simulink model "uartDemo"  (R2023a)
settings: Solver=ode4  StartTime=0.0  StopTime=0.011  FixedStep=0.01  RelTol=1e-3
libraries: simulink x10, instrumentseriallib x4, slrealtimeutilitieslib x2, svdutilitieslib x1
settings Model: Creator=zhuxh  LastModifiedBy=zqinghua
settings SolverCC: AlgebraicLoopSolver=TrustRegion
settings DebuggingCC: ArithmeticOperatorsInVariantConditions=warning
settings SFSimCC: CustomCodeUndefinedFunction=UseInterfaceOnly
settings CodeAppCC: StateflowObjectComments=on

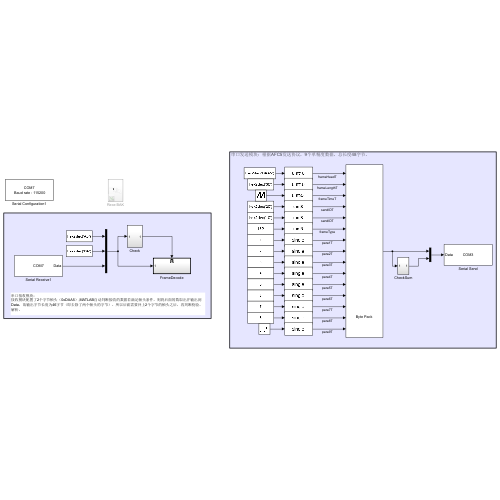
[thumbnail: Simulink's stored preview of the top-level diagram]
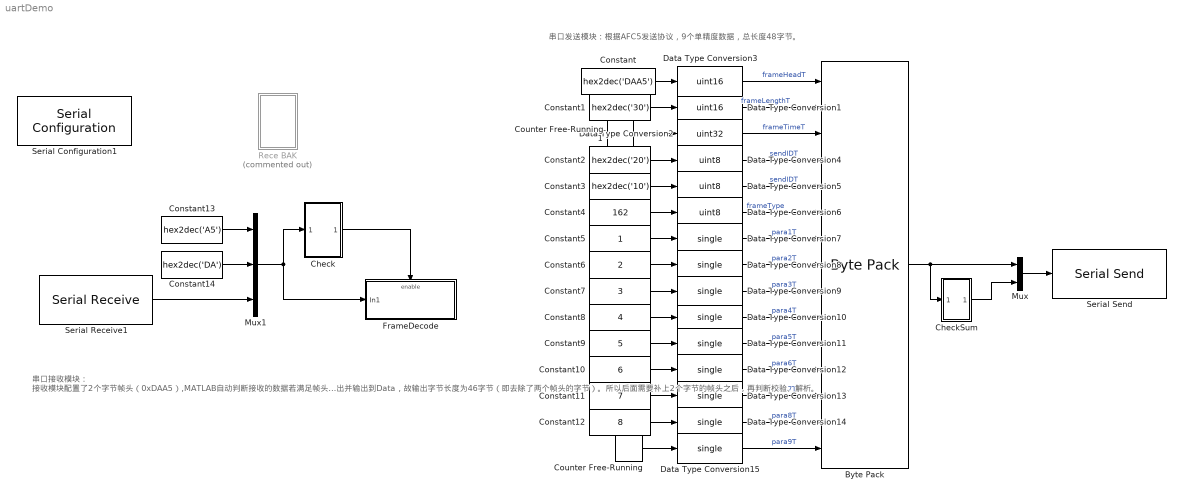
== system uartDemo ==
  note: 串口发送模块：根据AFC5发送协议，9个单精度数据，总长度48字节。
  note: 串口接收模块：
      | 接收模块配置了2个字节帧头（0xDAA5）,MATLAB自动判断接收的数据若满足帧头条件，则将后面的数取出并输出到Data，故输出字节长度为46字节（即去除了两个帧头的字节）。所以后面需要补上2个字节的帧头之后，再判断校验、解析。
  Byte Pack : svdutilitieslib/Byte Pack  maskPackedDataType=uint8  datatypes={'uint16','uint16','uint32','uint8','uint8','uint8','single','single','single','single','single','single','single','single','single'}  byteAlign=1  blockPlatform=tic2000
      settings: LibrarySourceBlock=c2000lib/Target Communication/Byte Pack
  Check : Subsystem
  CheckSum : Subsystem
  Constant : Constant  Value=hex2dec('DAA5')  SampleTime=-1
  Constant1 : Constant  Value=hex2dec('30')  SampleTime=-1
  Constant10 : Constant  Value=6  SampleTime=-1
  Constant11 : Constant  Value=7  SampleTime=-1
  Constant12 : Constant  Value=8  SampleTime=-1
  Constant13 : Constant  Value=hex2dec('A5')  OutDataTypeStr=uint8  SampleTime=-1
  Constant14 : Constant  Value=hex2dec('DA')  OutDataTypeStr=uint8  SampleTime=-1
  Constant2 : Constant  Value=hex2dec('20')  SampleTime=-1
  Constant3 : Constant  Value=hex2dec('10')  SampleTime=-1
  Constant4 : Constant  Value=162  SampleTime=-1
  Constant5 : Constant  SampleTime=-1
  Constant6 : Constant  Value=2  SampleTime=-1
  Constant7 : Constant  Value=3  SampleTime=-1
  Constant8 : Constant  Value=4  SampleTime=-1
  Constant9 : Constant  Value=5  SampleTime=-1
  Counter Free-Running : simulink/Sources/Counter Free-Running  NumBits=32  tsamp=-1
  Counter Free-Running1 : simulink/Sources/Counter Free-Running  NumBits=32  tsamp=-1
  Data Type Conversion1 : DataTypeConversion  OutDataTypeStr=uint16  SaturateOnIntegerOverflow=off  RndMeth=Floor
  Data Type Conversion{7..15} (9 alike) : DataTypeConversion  OutDataTypeStr=single  SaturateOnIntegerOverflow=off  RndMeth=Floor
  Data Type Conversion2 : DataTypeConversion  OutDataTypeStr=uint32  SaturateOnIntegerOverflow=off  RndMeth=Floor
  Data Type Conversion3 : DataTypeConversion  OutDataTypeStr=uint16  SaturateOnIntegerOverflow=off  RndMeth=Floor
  Data Type Conversion4 : DataTypeConversion  OutDataTypeStr=uint8  SaturateOnIntegerOverflow=off  RndMeth=Floor
  Data Type Conversion5 : DataTypeConversion  OutDataTypeStr=uint8  SaturateOnIntegerOverflow=off  RndMeth=Floor
  Data Type Conversion6 : DataTypeConversion  OutDataTypeStr=uint8  SaturateOnIntegerOverflow=off  RndMeth=Floor
  FrameDecode : Subsystem  TreatAsAtomicUnit=on
  Mux : Mux  Inputs=2
  Mux1 : Mux  Inputs=3
  Rece BAK : Subsystem  Commented=on
  Serial Configuration1 : instrumentseriallib/Serial Configuration  Priority=-200000  PortSel=COM7  Port=COM7  ComPort=COM7  BaudRate=115200  DataBits=8  Parity=none  StopBits=1  ByteOrder=little-endian  FlowControl=none  Timeout=10  SimulateUsing=Interpreted execution  BlockInModel=on  aMode=1
  Serial Receive1 : instrumentseriallib/Serial Receive  Priority=1  PortSel=COM7  Port=COM7  ComPort=COM7  DataType=uint8  SaveDataType=uint8  ToggleHeader=on  Header=[hex2dec('DA') hex2dec('A5')]  ToggleTerminator=off  Terminator=<none>  CustomTerminator=[]  InputFormat=Column major  ToggleDataSize=on  DataSize=46  EnableBlockingMode=on  ActionDataUnavailable=Output last received value  ActionWhenDataUnavailable=Output last received value  CustomValue=0  SampleTime=-1  SimulateUsing=Interpreted execution  BlockInModel=on  aMode=1
  Serial Send : instrumentseriallib/Serial Send  Priority=1  PortSel=COM3  Port=COM3  ComPort=COM3  Header=[]  Terminator=<none>  CustomTerminator=[]  EnableBlockingMode=on  SimulateUsing=Interpreted execution  BlockInModel=on  aMode=1
  wires:
  Data Type Conversion4/1 -> Byte Pack/4  "sendIDT"
  Data Type Conversion5/1 -> Byte Pack/5  "sendIDT"
  Data Type Conversion8/1 -> Byte Pack/8  "para2T"
  Data Type Conversion3/1 -> Byte Pack/1  "frameHeadT"
  Constant5/1 -> Data Type Conversion7/1
  Constant8/1 -> Data Type Conversion10/1
  Constant6/1 -> Data Type Conversion8/1
  Data Type Conversion11/1 -> Byte Pack/11  "para5T"
  Constant11/1 -> Data Type Conversion13/1
  Data Type Conversion10/1 -> Byte Pack/10  "para4T"
  Constant10/1 -> Data Type Conversion12/1
  Constant7/1 -> Data Type Conversion9/1
  Data Type Conversion7/1 -> Byte Pack/7  "para1T"
  Constant2/1 -> Data Type Conversion4/1
  Counter Free-Running1/1 -> Data Type Conversion2/1
  Mux/1 -> Serial Send/1
  Data Type Conversion2/1 -> Byte Pack/3  "frameTimeT"
  Counter Free-Running/1 -> Data Type Conversion15/1
  Data Type Conversion13/1 -> Byte Pack/13  "para7T"
  Data Type Conversion6/1 -> Byte Pack/6  "frameType"
  Data Type Conversion9/1 -> Byte Pack/9  "para3T"
  Constant/1 -> Data Type Conversion3/1
  Constant12/1 -> Data Type Conversion14/1
  Constant9/1 -> Data Type Conversion11/1
  CheckSum/1(Out1) -> Mux/2
  Data Type Conversion12/1 -> Byte Pack/12  "para6T"
  Constant4/1 -> Data Type Conversion6/1
  Data Type Conversion15/1 -> Byte Pack/15  "para9T"
  Constant1/1 -> Data Type Conversion1/1
  Constant3/1 -> Data Type Conversion5/1
  Data Type Conversion14/1 -> Byte Pack/14  "para8T"
  Byte Pack/1 -> CheckSum/1(In1), Mux/1
  Data Type Conversion1/1 -> Byte Pack/2  "frameLengthT"
  Serial Receive1/1 -> Mux1/3
  Constant13/1 -> Mux1/1
  Constant14/1 -> Mux1/2
  Mux1/1 -> Check/1(In1), FrameDecode/1(In1)
  Check/1(Out1) -> FrameDecode/Enable

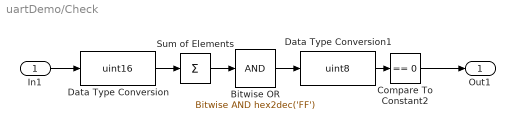
== system uartDemo/Check ==
  In1 : Inport
  Bitwise OR : simulink/Logic and Bit Operations/Bitwise Operator  logicop=AND  UseBitMask=on  BitMask=hex2dec('FF')  BitMaskRealWorld=Stored Integer
  Compare To Constant2 : simulink/Logic and Bit Operations/Compare To Constant  relop===  const=0  OutDataTypeStr=boolean
  Data Type Conversion : DataTypeConversion  OutDataTypeStr=uint16  SaturateOnIntegerOverflow=off  RndMeth=Floor
  Data Type Conversion1 : DataTypeConversion  OutDataTypeStr=uint8  SaturateOnIntegerOverflow=off  RndMeth=Floor
  Sum of Elements : Sum  Inputs=+
  Out1 : Outport
  wires:
  Compare To Constant2/1 -> Out1/1
  Sum of Elements/1 -> Bitwise OR/1
  Bitwise OR/1 -> Data Type Conversion1/1
  Data Type Conversion/1 -> Sum of Elements/1
  Data Type Conversion1/1 -> Compare To Constant2/1
  In1/1 -> Data Type Conversion/1

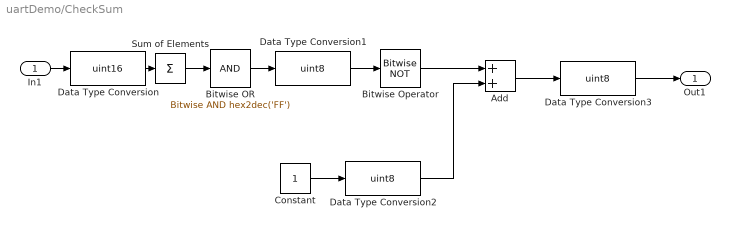
== system uartDemo/CheckSum ==
  In1 : Inport
  Add : Sum
  Bitwise Operator : simulink/Logic and Bit Operations/Bitwise Operator  logicop=NOT  UseBitMask=off  BitMask=bin2dec('11011001')  BitMaskRealWorld=Stored Integer
  Bitwise OR : simulink/Logic and Bit Operations/Bitwise Operator  logicop=AND  UseBitMask=on  BitMask=hex2dec('FF')  BitMaskRealWorld=Stored Integer
  Constant : Constant
  Data Type Conversion : DataTypeConversion  OutDataTypeStr=uint16  SaturateOnIntegerOverflow=off  RndMeth=Floor
  Data Type Conversion1 : DataTypeConversion  OutDataTypeStr=uint8  SaturateOnIntegerOverflow=off  RndMeth=Floor
  Data Type Conversion2 : DataTypeConversion  OutDataTypeStr=uint8  SaturateOnIntegerOverflow=off  RndMeth=Floor
  Data Type Conversion3 : DataTypeConversion  OutDataTypeStr=uint8  SaturateOnIntegerOverflow=off  RndMeth=Floor
  Sum of Elements : Sum  Inputs=+
  Out1 : Outport
  wires:
  Data Type Conversion3/1 -> Out1/1
  Sum of Elements/1 -> Bitwise OR/1
  Bitwise OR/1 -> Data Type Conversion1/1
  Data Type Conversion/1 -> Sum of Elements/1
  Data Type Conversion1/1 -> Bitwise Operator/1
  In1/1 -> Data Type Conversion/1
  Bitwise Operator/1 -> Add/1
  Constant/1 -> Data Type Conversion2/1
  Data Type Conversion2/1 -> Add/2
  Add/1 -> Data Type Conversion3/1

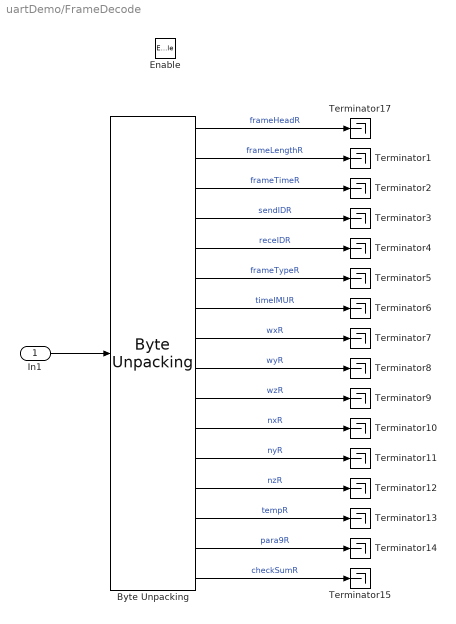
== system uartDemo/FrameDecode ==
  In1 : Inport
  Enable : EnablePort
  "Byte Unpacking " : slrealtimeutilitieslib/Byte Unpacking  MaskUnpackedDataTypes={'uint16','uint16','uint32','uint8','uint8','uint8','single','single','single','single','single','single','single','single','single','uint8'}  MaskUnpackedDataSizes={1,1,1,1,1,1,1,1,1,1,1,1,1,1,1,1}  MaskAlignment=1
  Terminator{1..15,17} (16 alike) : Terminator
  wires:
  "Byte Unpacking "/11 -> Terminator10/1  "nxR"
  "Byte Unpacking "/1 -> Terminator17/1  "frameHeadR"
  "Byte Unpacking "/8 -> Terminator7/1  "wxR"
  "Byte Unpacking "/13 -> Terminator12/1  "nzR"
  "Byte Unpacking "/5 -> Terminator4/1  "receIDR"
  "Byte Unpacking "/14 -> Terminator13/1  "tempR"
  "Byte Unpacking "/6 -> Terminator5/1  "frameTypeR"
  "Byte Unpacking "/3 -> Terminator2/1  "frameTimeR"
  "Byte Unpacking "/2 -> Terminator1/1  "frameLengthR"
  "Byte Unpacking "/16 -> Terminator15/1  "checkSumR"
  "Byte Unpacking "/15 -> Terminator14/1  "para9R"
  "Byte Unpacking "/12 -> Terminator11/1  "nyR"
  "Byte Unpacking "/10 -> Terminator9/1  "wzR"
  "Byte Unpacking "/9 -> Terminator8/1  "wyR"
  "Byte Unpacking "/7 -> Terminator6/1  "timeIMUR"
  "Byte Unpacking "/4 -> Terminator3/1  "sendIDR"
  In1/1 -> "Byte Unpacking "/1

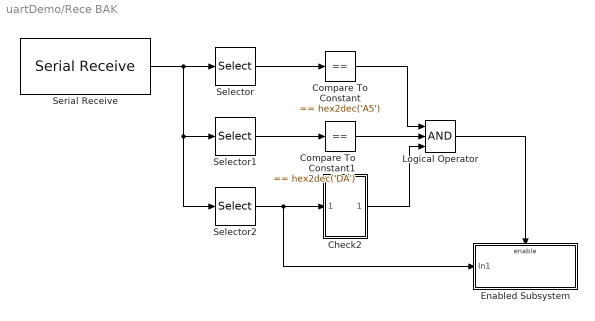
== system uartDemo/Rece BAK ==
  Check2 : Subsystem
  Compare To Constant : simulink/Logic and Bit Operations/Compare To Constant  relop===  const=hex2dec('A5')  OutDataTypeStr=boolean
  Compare To Constant1 : simulink/Logic and Bit Operations/Compare To Constant  relop===  const=hex2dec('DA')  OutDataTypeStr=boolean
  Enabled Subsystem : Subsystem  TreatAsAtomicUnit=on
  Logical Operator : Logic  Inputs=3  AllPortsSameDT=off  OutDataTypeStr=boolean
  Selector : Selector  InputPortWidth=48  IndexOptions=Index vector (dialog)  Indices=[1]  OutputSizes=1
  Selector1 : Selector  InputPortWidth=48  IndexOptions=Index vector (dialog)  Indices=[2]  OutputSizes=1
  Selector2 : Selector  InputPortWidth=48  IndexOptions=Index vector (dialog)  Indices=[1:48]  OutputSizes=1
  Serial Receive : instrumentseriallib/Serial Receive  Priority=1  PortSel=COM3  Port=COM3  ComPort=COM3  DataType=uint8  SaveDataType=uint8  ToggleHeader=off  Header=[]  ToggleTerminator=off  Terminator=<none>  CustomTerminator=[]  InputFormat=Column major  ToggleDataSize=on  DataSize=48  EnableBlockingMode=on  ActionDataUnavailable=Output last received value  ActionWhenDataUnavailable=Output last received value  CustomValue=0  SampleTime=-1  SimulateUsing=Interpreted execution  BlockInModel=on  aMode=1
  wires:
  Logical Operator/1 -> Enabled Subsystem/Enable
  Serial Receive/1 -> Selector/1, Selector2/1, Selector1/1
  Check2/1(Out1) -> Logical Operator/3
  Selector1/1 -> Compare To Constant1/1
  Selector/1 -> Compare To Constant/1
  Compare To Constant/1 -> Logical Operator/1
  Compare To Constant1/1 -> Logical Operator/2
  Selector2/1 -> Enabled Subsystem/1(In1), Check2/1(In1)

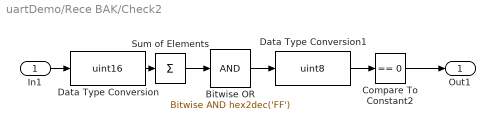
== system uartDemo/Rece BAK/Check2 ==
  In1 : Inport
  Bitwise OR : simulink/Logic and Bit Operations/Bitwise Operator  logicop=AND  UseBitMask=on  BitMask=hex2dec('FF')  BitMaskRealWorld=Stored Integer
  Compare To Constant2 : simulink/Logic and Bit Operations/Compare To Constant  relop===  const=0  OutDataTypeStr=boolean
  Data Type Conversion : DataTypeConversion  OutDataTypeStr=uint16  SaturateOnIntegerOverflow=off  RndMeth=Floor
  Data Type Conversion1 : DataTypeConversion  OutDataTypeStr=uint8  SaturateOnIntegerOverflow=off  RndMeth=Floor
  Sum of Elements : Sum  Inputs=+
  Out1 : Outport
  wires:
  Compare To Constant2/1 -> Out1/1
  Sum of Elements/1 -> Bitwise OR/1
  Bitwise OR/1 -> Data Type Conversion1/1
  Data Type Conversion/1 -> Sum of Elements/1
  Data Type Conversion1/1 -> Compare To Constant2/1
  In1/1 -> Data Type Conversion/1

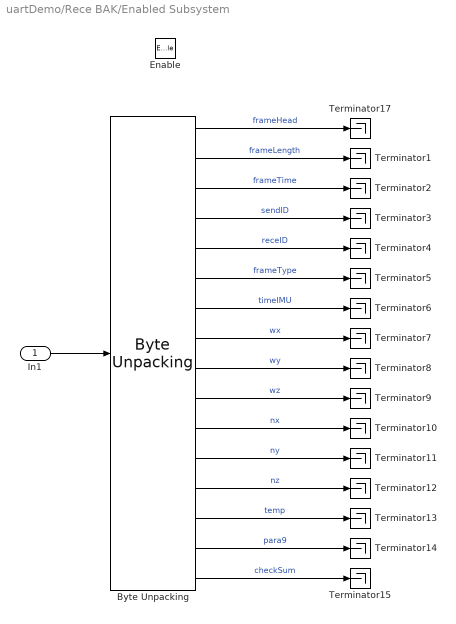
== system uartDemo/Rece BAK/Enabled Subsystem ==
  In1 : Inport
  Enable : EnablePort
  "Byte Unpacking " : slrealtimeutilitieslib/Byte Unpacking  MaskUnpackedDataTypes={'uint16','uint16','uint32','uint8','uint8','uint8','single','single','single','single','single','single','single','single','single','uint8'}  MaskUnpackedDataSizes={1,1,1,1,1,1,1,1,1,1,1,1,1,1,1,1}  MaskAlignment=1
  Terminator{1..15,17} (16 alike) : Terminator
  wires:
  "Byte Unpacking "/11 -> Terminator10/1  "nx"
  "Byte Unpacking "/1 -> Terminator17/1  "frameHead"
  "Byte Unpacking "/8 -> Terminator7/1  "wx"
  "Byte Unpacking "/13 -> Terminator12/1  "nz"
  "Byte Unpacking "/5 -> Terminator4/1  "receID"
  "Byte Unpacking "/14 -> Terminator13/1  "temp"
  "Byte Unpacking "/6 -> Terminator5/1  "frameType"
  "Byte Unpacking "/3 -> Terminator2/1  "frameTime"
  "Byte Unpacking "/2 -> Terminator1/1  "frameLength"
  "Byte Unpacking "/16 -> Terminator15/1  "checkSum"
  "Byte Unpacking "/15 -> Terminator14/1  "para9"
  "Byte Unpacking "/12 -> Terminator11/1  "ny"
  "Byte Unpacking "/10 -> Terminator9/1  "wz"
  "Byte Unpacking "/9 -> Terminator8/1  "wy"
  "Byte Unpacking "/7 -> Terminator6/1  "timeIMU"
  "Byte Unpacking "/4 -> Terminator3/1  "sendID"
  In1/1 -> "Byte Unpacking "/1
